simulink model "rocket_roll_model"  (R2026b)
settings: Solver=ode4  StopTime=5  FixedStep=1e-4
PreLoadFcn:
  | J_v = 0.0125; J_w = 0.002535; b = 0.002; Kp = 369.82; Ki = 616.37; Kd = 73.18;
InitFcn:
  | J_v = 0.0125; J_w = 0.002535; b = 0.002; Kp = 369.82; Ki = 616.37; Kd = 73.18;
settings Model: Creator=Nirmal Krishna P  LastModifiedBy=Nirmal Krishna P

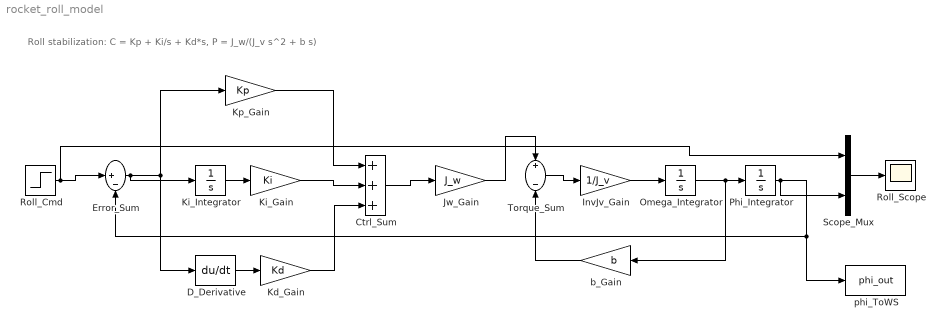
== system rocket_roll_model ==
  note: Roll stabilization: C = Kp + Ki/s + Kd*s, P = J_w/(J_v s^2 + b s)
  Ctrl_Sum : Sum  Inputs=+++
  D_Derivative : Derivative
  Error_Sum : Sum  Inputs=|+-
  InvJv_Gain : Gain  Gain=1/J_v
  Jw_Gain : Gain  Gain=J_w
  Kd_Gain : Gain  Gain=Kd
  Ki_Gain : Gain  Gain=Ki
  Ki_Integrator : Integrator
  Kp_Gain : Gain  Gain=Kp
  Omega_Integrator : Integrator
  Phi_Integrator : Integrator
  Roll_Cmd : Step  Time=0  SampleTime=0
  Roll_Scope : Scope
  Scope_Mux : Mux  Inputs=2
  Torque_Sum : Sum  Inputs=+-
  b_Gain : Gain  Gain=b
  phi_ToWS : ToWorkspace  VariableName=phi_out  SampleTime=-1
  wires:
  Roll_Cmd/1 -> Error_Sum/1, Scope_Mux/1
  Error_Sum/1 -> Kp_Gain/1, D_Derivative/1, Ki_Integrator/1
  Ki_Integrator/1 -> Ki_Gain/1
  D_Derivative/1 -> Kd_Gain/1
  Kp_Gain/1 -> Ctrl_Sum/1
  Ki_Gain/1 -> Ctrl_Sum/2
  Kd_Gain/1 -> Ctrl_Sum/3
  Ctrl_Sum/1 -> Jw_Gain/1
  Jw_Gain/1 -> Torque_Sum/1
  Torque_Sum/1 -> InvJv_Gain/1
  InvJv_Gain/1 -> Omega_Integrator/1
  Omega_Integrator/1 -> Phi_Integrator/1, b_Gain/1
  b_Gain/1 -> Torque_Sum/2
  Phi_Integrator/1 -> Error_Sum/2, phi_ToWS/1, Scope_Mux/2
  Scope_Mux/1 -> Roll_Scope/1
